simulink model "Lab2SimN"  (R2025b)
settings: Solver=VariableStepAuto  StartTime=0.0  StopTime=48*3600  RelTol=1e-3
values from neighbouring files (symbols this model uses):
  k = 1/580    (= 0.00172413793103)    [Lab2.m]    (also in Lab2N.m)
  P = 35960    [Lab2.m]    (also in Lab2N.m = 30740)
  Pz = Ub*(Tu+Tzz)    (= 13340)    [Lab2N.m]
  Q = 937500    [Lab2.m]    (also in Lab2N.m)
  T = Q/580    (= 1616.37931034)    [Lab2.m]    (also in Lab2N.m)
  Tz = 30    [Lab2N.m]
  Tzz = 0    [Lab2N.m]
  Ub = (4*Us)+Uo    (= 580)    [Lab2N.m]
settings Model: PacingRate=0.079000  Creator=dorian  LastModifiedBy=dorian

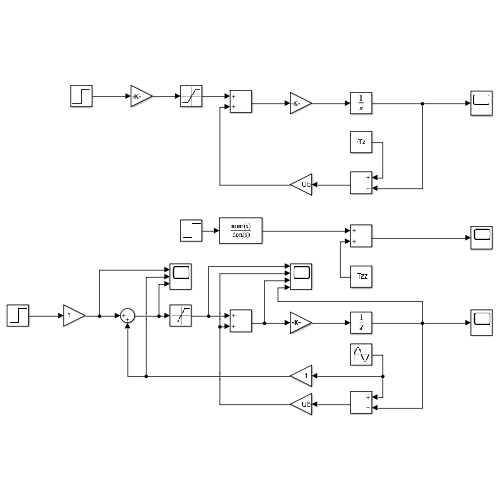
[thumbnail: Simulink's stored preview of the top-level diagram]
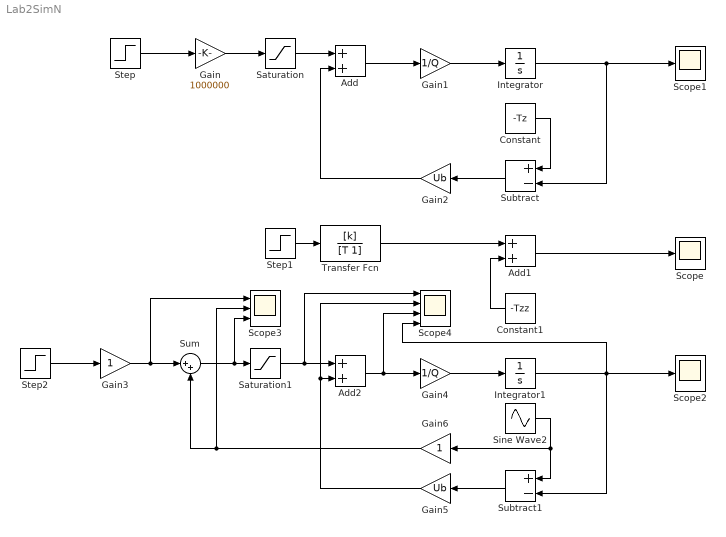
== system Lab2SimN ==
  Add : Sum
  Add1 : Sum
  Add2 : Sum
  Constant : Constant  Value=-Tz
  Constant1 : Constant  Value=-Tzz
  Gain : Gain  Gain=1000000
  Gain1 : Gain  Gain=1/Q
  Gain2 : Gain  Gain=Ub
  Gain3 : Gain
  Gain4 : Gain  Gain=1/Q
  Gain5 : Gain  Gain=Ub
  Gain6 : Gain
  Integrator : Integrator
  Integrator1 : Integrator
  Saturation : Saturate  UpperLimit=P  LowerLimit=0
  Saturation1 : Saturate  UpperLimit=P
  Scope : Scope
      settings: ActiveDisplayYMinimum=-1  ActiveDisplayYMaximum=1
  Scope1 : Scope
      settings: ActiveDisplayYMinimum=-2.8958735424517581  ActiveDisplayYMaximum=25.877319282494639
  Scope2 : Scope
      settings: ActiveDisplayYMinimum=-3.5121037927135488  ActiveDisplayYMaximum=31.455382568875436  DataLoggingVariableName=ScopeData2
  Scope3 : Scope  NumInputPorts=3
      settings: ActiveDisplayYMinimum=-8217.000343076088  ActiveDisplayYMaximum=38957.000343076084  DataLoggingVariableName=ScopeData3
  Scope4 : Scope  NumInputPorts=4
      settings: ActiveDisplayYMinimum=-57288.433597162664  ActiveDisplayYMaximum=46260.715056065761  DataLoggingVariableName=ScopeData4
  Sine Wave2 : Sin  Amplitude=5  Bias=-Tz  Frequency=(pi*2)/(24*3600)  SampleTime=0
  Step : Step  After=24*3600  SampleTime=0
  Step1 : Step  After=Pz  SampleTime=0
  Step2 : Step  After=P  SampleTime=0
  Subtract : Sum  Inputs=+-
  Subtract1 : Sum  Inputs=+-
  Sum : Sum  Inputs=|++
  Transfer Fcn : TransferFcn  Numerator=[k]  Denominator=[T 1]
  wires:
  Step/1 -> Gain/1
  Add/1 -> Gain1/1
  Gain1/1 -> Integrator/1
  Integrator/1 -> Scope1/1, Subtract/2
  Constant/1 -> Subtract/1
  Gain/1 -> Saturation/1
  Saturation/1 -> Add/1
  Subtract/1 -> Gain2/1
  Gain2/1 -> Add/2
  Add1/1 -> Scope/1
  Constant1/1 -> Add1/2
  Step1/1 -> Transfer Fcn/1
  Transfer Fcn/1 -> Add1/1
  Gain5/1 -> Scope4/2, Add2/2
  Gain4/1 -> Integrator1/1
  Subtract1/1 -> Gain5/1
  Add2/1 -> Scope4/3, Gain4/1
  Integrator1/1 -> Scope4/4, Subtract1/2, Scope2/1
  Sine Wave2/1 -> Gain6/1, Subtract1/1
  Saturation1/1 -> Scope4/1, Add2/1
  Sum/1 -> Scope3/3, Saturation1/1
  Gain3/1 -> Scope3/1, Sum/1
  Step2/1 -> Gain3/1
  Gain6/1 -> Scope3/2, Sum/2
